simulink model "hamming_enc_sl"  (R2026b)
settings: Solver=FixedStepDiscrete  StopTime=111  FixedStep=1
libraries: simulink x2
settings Model: Creator=INS NAWEL  LastModifiedBy=INS NAWEL

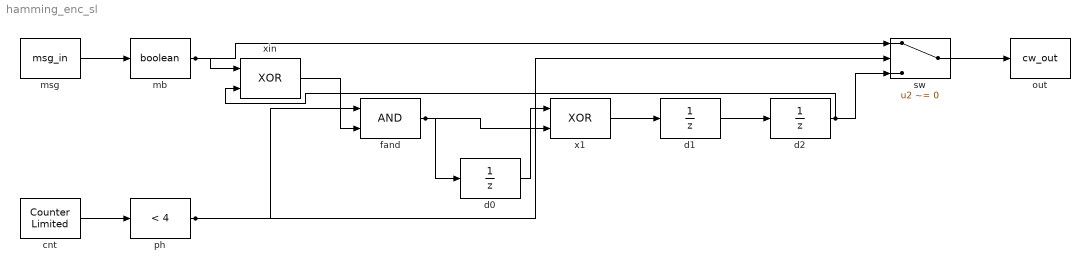
== system hamming_enc_sl ==
  cnt : simulink/Sources/Counter Limited  uplimit=6  tsamp=1
  d0 : UnitDelay
  d1 : UnitDelay
  d2 : UnitDelay
  fand : Logic  AllPortsSameDT=off  OutDataTypeStr=boolean
  mb : DataTypeConversion  OutDataTypeStr=boolean  SaturateOnIntegerOverflow=off  RndMeth=Floor
  msg : FromWorkspace  VariableName=msg_in  SampleTime=1
  out : ToWorkspace  VariableName=cw_out  SampleTime=1
  ph : simulink/Logic and Bit Operations/Compare To Constant  relop=<  const=4  OutDataTypeStr=boolean
  sw : Switch  Criteria=u2 ~= 0  SaturateOnIntegerOverflow=off  InputSameDT=off
  x1 : Logic  Operator=XOR  AllPortsSameDT=off  OutDataTypeStr=boolean
  xin : Logic  Operator=XOR  AllPortsSameDT=off  OutDataTypeStr=boolean
  wires:
  msg/1 -> mb/1
  cnt/1 -> ph/1
  mb/1 -> xin/1, sw/1
  d2/1 -> xin/2, sw/3
  ph/1 -> fand/1, sw/2
  xin/1 -> fand/2
  fand/1 -> d0/1, x1/2
  d0/1 -> x1/1
  x1/1 -> d1/1
  d1/1 -> d2/1
  sw/1 -> out/1
